simulink model "mars_rover_test_harness_chassis"  (R2025a)
settings: Solver=ode23t  StartTime=0.0  StopTime=30  FixedStep=1e-10  MaxStep=1e-1  RelTol=1e-3  AbsTol=1e-3  EnableMultiTasking=on
undefined symbols (not defined in the file): arm_q0, Control, L1, L2, L3, LS1, LS3, R1, R2, R3, Rover, RS1, RS3, X, Y, Z
libraries: sm_lib x119, nesl_utility x99, fl_lib x85, sdl_lib x20, ee_lib x10, mars_rover_lib x8, simulink x5, slpidlib x3, batteryecm_lib x2
(part 2 of 8)

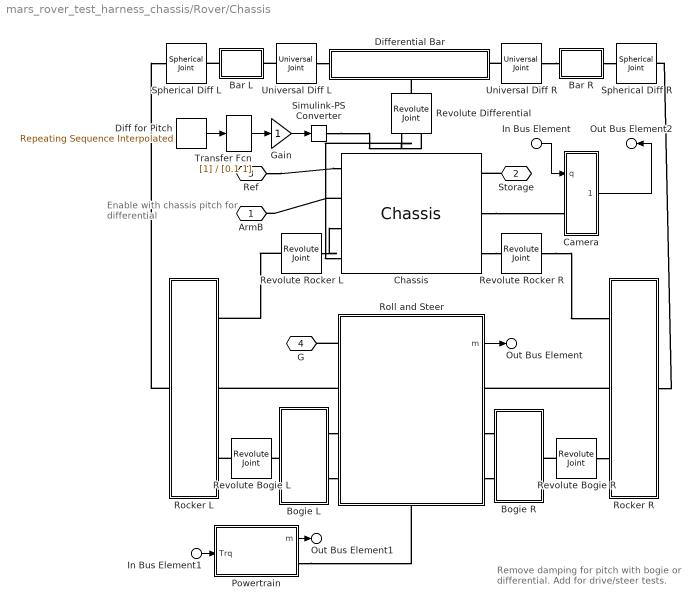
== system mars_rover_test_harness_chassis/Rover/Chassis ==
  note: Enable with chassis pitch for differential
  note: Remove damping for pitch with bogie or differential. Add for drive/steer tests.
  In Bus Element1 : Inport  PortName=Ctrl
  In Bus Element : Inport  PortName=Ctrl  Element=Camera
  Bar L : Subsystem
  Bar R : Subsystem
  Bogie L : Subsystem
      mask Display: image('mars_rover_terrain_chassis_bogiel.png');
  Bogie R : Subsystem
      mask Display: image('mars_rover_terrain_chassis_bogier.png');
  Camera : Subsystem
      mask Display: image('mars_rover_terrain_chassis_camera.png')
  Chassis : mars_rover_lib/Chassis  body_opc=1
  Diff for Pitch : simulink/Sources/Repeating Sequence Interpolated  OutValues=-0.5*[0 0 1 1 0 0 -1 -1 0 0]*5*pi/180.'  TimeValues=[0 2 4 7 9 11 13 16 18 20].'  LookUpMeth=Interpolation-Use End Values  tsamp=0.01  OutMin=[]  OutMax=[]  OutDataTypeStr=double  OutputDataTypeScalingMode=double  OutDataType=fixdt(0,8)  OutScaling=2^-10
  Differential Bar : Subsystem
      settings: PortSchema="{\"entries\":[{\"content\":{\"sides\":[{\"content\":{\"connectorIds\":[\"LConn1\"]},\"type\":\"ConnectorPlacement.EquallySpacedRectSide\",\"uuid\":\"221cdbde-9b85-4491-b488-ab21b8b80dc6\"},{\"content\":{\"connectorIds\":[\"RConn1\"],\"side\":\"RIGHT\"},\"type\":\"ConnectorPlacement.EquallySpacedRectSide\",\"uuid\":\"70e1e311-dd19-4389-b9b6-0ef8a1761d4a\"},{\"content\":{\"connectorIds\":[],\"side\":\"TOP\"},\"type\":\"ConnectorPlacement.EquallySpacedRectSide\",\"uuid\":\"5e164d53-108c-4bd4-88ac-8f7d3d652b3e\"},{\"content\":{\"connectorIds\":[\"RConn2\"],\"side\":\"BOTTOM\"},\"type\":\"ConnectorPlacement.EquallySpacedRectSide\",\"uuid\":\"f6e2e044-5d94-4f88-a007-0ec3cd9ea455\"}]},\"type\":\"ConnectorPlacement.EquallySpacedConnector\",\"uuid\":\"e7d2f355-3189-4eee-a2bf-989eae5d727a\"}],\"packageUris\":[\"http://schema.mathworks.com/mf0/Connector/R2020b\"],\"version\":\"1.0\"}"
      mask Display: image('mars_rover_terrain_chassis_diffarm.png');
  Gain : Gain
  Powertrain : Subsystem  Variant=on  VariantControlMode=label  VariantControl=Choice  LabelModeActiveChoice=Ideal  mask{popup_powertrain=Ideal}
      mask prompts: popup_powertrain "Powertrain Model"
      mask init:
      | set_param(gcb,'LabelModeActiveChoice',get_param(gcb,'popup_powertrain'));
      settings: AttributesFormatString=%<LabelModeActiveChoice>
      mask TypeOptions popup_powertrain: Ideal | Electrical
  Revolute Bogie L : sm_lib/Joints/Revolute Joint  JointMode=Normal  CompositeWrenchDir=FollowerOnBase  CompositeWrenchFrame=BaseFrame  SenseConstraintForce=off  SenseConstraintTorque=off  SenseTotalForce=off  SenseTotalTorque=off  PositionTargetSpecify=off  PositionTargetPriority=High  PositionTargetValue=0  PositionTargetValueUnits=deg  VelocityTargetSpecify=off  VelocityTargetPriority=High  VelocityTargetValue=0  VelocityTargetValueUnits=deg/s  EquilibriumPosition=0  EquilibriumPositionUnits=deg  SpringStiffness=0  SpringStiffnessUnits=N*m/deg  DampingCoefficient=1e3*0  DampingCoefficientUnits=N*m/(deg/s)  LowerLimitSpecify=off  LowerLimitBound=-90  LowerLimitBoundUnits=deg  LowerLimitStiffness=1e4  LowerLimitStiffnessUnits=N*m/deg  LowerLimitDamping=10  LowerLimitDampingUnits=N*m/(deg/s)  LowerLimitTransitionRegionWidth=0.1  LowerLimitTransitionRegionWidthUnits=deg  UpperLimitSpecify=off  UpperLimitBound=90  UpperLimitBoundUnits=deg  UpperLimitStiffness=1e4  UpperLimitStiffnessUnits=N*m/deg  UpperLimitDamping=10  UpperLimitDampingUnits=N*m/(deg/s)  UpperLimitTransitionRegionWidth=0.1  UpperLimitTransitionRegionWidthUnits=deg  TorqueActuationMode=NoTorque  MotionActuationMode=ComputedMotion  SensePosition=off  SenseVelocity=off  SenseAcceleration=off  SenseTorqueForce=off  SenseLowerLimitTorqueForce=off  SenseUpperLimitTorqueForce=off
  Revolute Bogie R : sm_lib/Joints/Revolute Joint  JointMode=Normal  CompositeWrenchDir=FollowerOnBase  CompositeWrenchFrame=BaseFrame  SenseConstraintForce=off  SenseConstraintTorque=off  SenseTotalForce=off  SenseTotalTorque=off  PositionTargetSpecify=off  PositionTargetPriority=High  PositionTargetValue=0  PositionTargetValueUnits=deg  VelocityTargetSpecify=off  VelocityTargetPriority=High  VelocityTargetValue=0  VelocityTargetValueUnits=deg/s  EquilibriumPosition=0  EquilibriumPositionUnits=deg  SpringStiffness=0  SpringStiffnessUnits=N*m/deg  DampingCoefficient=1e3*0  DampingCoefficientUnits=N*m/(deg/s)  LowerLimitSpecify=off  LowerLimitBound=-90  LowerLimitBoundUnits=deg  LowerLimitStiffness=1e4  LowerLimitStiffnessUnits=N*m/deg  LowerLimitDamping=10  LowerLimitDampingUnits=N*m/(deg/s)  LowerLimitTransitionRegionWidth=0.1  LowerLimitTransitionRegionWidthUnits=deg  UpperLimitSpecify=off  UpperLimitBound=90  UpperLimitBoundUnits=deg  UpperLimitStiffness=1e4  UpperLimitStiffnessUnits=N*m/deg  UpperLimitDamping=10  UpperLimitDampingUnits=N*m/(deg/s)  UpperLimitTransitionRegionWidth=0.1  UpperLimitTransitionRegionWidthUnits=deg  TorqueActuationMode=NoTorque  MotionActuationMode=ComputedMotion  SensePosition=off  SenseVelocity=off  SenseAcceleration=off  SenseTorqueForce=off  SenseLowerLimitTorqueForce=off  SenseUpperLimitTorqueForce=off
  Revolute Differential : sm_lib/Joints/Revolute Joint  JointMode=Normal  CompositeWrenchDir=FollowerOnBase  CompositeWrenchFrame=BaseFrame  SenseConstraintForce=off  SenseConstraintTorque=off  SenseTotalForce=off  SenseTotalTorque=off  PositionTargetSpecify=off  PositionTargetPriority=High  PositionTargetValue=45  PositionTargetValueUnits=deg  VelocityTargetSpecify=off  VelocityTargetPriority=High  VelocityTargetValue=1000  VelocityTargetValueUnits=deg/s  EquilibriumPosition=0  EquilibriumPositionUnits=deg  SpringStiffness=0  SpringStiffnessUnits=N*m/deg  DampingCoefficient=1e-3  DampingCoefficientUnits=N*m/(rad/s)  LowerLimitSpecify=off  LowerLimitBound=-90  LowerLimitBoundUnits=deg  LowerLimitStiffness=1e4  LowerLimitStiffnessUnits=N*m/deg  LowerLimitDamping=10  LowerLimitDampingUnits=N*m/(deg/s)  LowerLimitTransitionRegionWidth=0.1  LowerLimitTransitionRegionWidthUnits=deg  UpperLimitSpecify=off  UpperLimitBound=90  UpperLimitBoundUnits=deg  UpperLimitStiffness=1e4  UpperLimitStiffnessUnits=N*m/deg  UpperLimitDamping=10  UpperLimitDampingUnits=N*m/(deg/s)  UpperLimitTransitionRegionWidth=0.1  UpperLimitTransitionRegionWidthUnits=deg  TorqueActuationMode=ComputedTorque  MotionActuationMode=InputMotion  SensePosition=off  SenseVelocity=off  SenseAcceleration=off  SenseTorqueForce=off  SenseLowerLimitTorqueForce=off  SenseUpperLimitTorqueForce=off
  Revolute Rocker L : sm_lib/Joints/Revolute Joint  JointMode=Normal  CompositeWrenchDir=FollowerOnBase  CompositeWrenchFrame=BaseFrame  SenseConstraintForce=off  SenseConstraintTorque=off  SenseTotalForce=off  SenseTotalTorque=off  PositionTargetSpecify=on  PositionTargetPriority=Low  PositionTargetValue=90  PositionTargetValueUnits=deg  VelocityTargetSpecify=off  VelocityTargetPriority=High  VelocityTargetValue=5  VelocityTargetValueUnits=deg/s  EquilibriumPosition=0  EquilibriumPositionUnits=deg  SpringStiffness=0  SpringStiffnessUnits=N*m/deg  DampingCoefficient=1e3  DampingCoefficientUnits=N*m/(rad/s)  LowerLimitSpecify=off  LowerLimitBound=-90  LowerLimitBoundUnits=deg  LowerLimitStiffness=1e4  LowerLimitStiffnessUnits=N*m/deg  LowerLimitDamping=10  LowerLimitDampingUnits=N*m/(deg/s)  LowerLimitTransitionRegionWidth=0.1  LowerLimitTransitionRegionWidthUnits=deg  UpperLimitSpecify=off  UpperLimitBound=90  UpperLimitBoundUnits=deg  UpperLimitStiffness=1e4  UpperLimitStiffnessUnits=N*m/deg  UpperLimitDamping=10  UpperLimitDampingUnits=N*m/(deg/s)  UpperLimitTransitionRegionWidth=0.1  UpperLimitTransitionRegionWidthUnits=deg  TorqueActuationMode=NoTorque  MotionActuationMode=ComputedMotion  SensePosition=off  SenseVelocity=off  SenseAcceleration=off  SenseTorqueForce=off  SenseLowerLimitTorqueForce=off  SenseUpperLimitTorqueForce=off
  Revolute Rocker R : sm_lib/Joints/Revolute Joint  JointMode=Normal  CompositeWrenchDir=FollowerOnBase  CompositeWrenchFrame=BaseFrame  SenseConstraintForce=off  SenseConstraintTorque=off  SenseTotalForce=off  SenseTotalTorque=off  PositionTargetSpecify=on  PositionTargetPriority=Low  PositionTargetValue=-90  PositionTargetValueUnits=deg  VelocityTargetSpecify=off  VelocityTargetPriority=High  VelocityTargetValue=5  VelocityTargetValueUnits=deg/s  EquilibriumPosition=0  EquilibriumPositionUnits=deg  SpringStiffness=0  SpringStiffnessUnits=N*m/deg  DampingCoefficient=1e3  DampingCoefficientUnits=N*m/(rad/s)  LowerLimitSpecify=off  LowerLimitBound=-90  LowerLimitBoundUnits=deg  LowerLimitStiffness=1e4  LowerLimitStiffnessUnits=N*m/deg  LowerLimitDamping=10  LowerLimitDampingUnits=N*m/(deg/s)  LowerLimitTransitionRegionWidth=0.1  LowerLimitTransitionRegionWidthUnits=deg  UpperLimitSpecify=off  UpperLimitBound=90  UpperLimitBoundUnits=deg  UpperLimitStiffness=1e4  UpperLimitStiffnessUnits=N*m/deg  UpperLimitDamping=10  UpperLimitDampingUnits=N*m/(deg/s)  UpperLimitTransitionRegionWidth=0.1  UpperLimitTransitionRegionWidthUnits=deg  TorqueActuationMode=NoTorque  MotionActuationMode=ComputedMotion  SensePosition=off  SenseVelocity=off  SenseAcceleration=off  SenseTorqueForce=off  SenseLowerLimitTorqueForce=off  SenseUpperLimitTorqueForce=off
  Rocker L : Subsystem
      mask Display: image('mars_rover_terrain_chassis_rockerl.png');
  Rocker R : Subsystem
      mask Display: image('mars_rover_terrain_chassis_rockerr.png');
  Roll and Steer : Subsystem
      settings: PortSchema="{\"entries\":[{\"content\":{\"sides\":[{\"content\":{\"connectorIds\":[\"LConn1\",\"LConn2\",\"LConn3\",\"LConn4\"]},\"type\":\"ConnectorPlacement.EquallySpacedRectSide\",\"uuid\":\"a6cfb551-8d36-4b7b-a27d-860438164ad5\"},{\"content\":{\"connectorIds\":[\"Out1\",\"RConn1\",\"RConn2\",\"RConn3\"],\"side\":\"RIGHT\"},\"type\":\"ConnectorPlacement.EquallySpacedRectSide\",\"uuid\":\"63cd4134-c970-4875-8139-e10b865c9d5a\"},{\"content\":{\"connectorIds\":[],\"side\":\"TOP\"},\"type\":\"ConnectorPlacement.EquallySpacedRectSide\",\"uuid\":\"731de0f8-cd01-497c-8464-7874165ef328\"},{\"content\":{\"connectorIds\":[\"RConn4\"],\"side\":\"BOTTOM\"},\"type\":\"ConnectorPlacement.EquallySpacedRectSide\",\"uuid\":\"7e28c2ad-ee21-4cfa-8326-dce39ed3da54\"}]},\"type\":\"ConnectorPlacement.EquallySpacedConnector\",\"uuid\":\"7cc269d8-0205-4cd4-bd76-499a6cc04585\"}],\"packageUris\":[\"http://schema.mathworks.com/mf0/Connector/R2020b\"],\"version\":\"1.0\"}"
      mask Display: image('mars_rover_terrain_rollandsteer.png');
  Simulink-PS Converter : nesl_utility/Simulink-PS Converter  PhysicalDomain=network_engine_domain  SubClassName=ps_input  LeftPortType=input  RightPortType=output  PseudoPeriodic=off  Frequencies=[]  NoiseDistribution=none  NoiseParameters=[]  Unit=1  AffineConversion=off  FilteringAndDerivatives=filter  SimscapeFilterOrder=2  InputFilterTimeConstant=0.01  UdotUserProvided=0
  Spherical Diff L : sm_lib/Joints/Spherical Joint  JointMode=Normal  CompositeWrenchDir=FollowerOnBase  CompositeWrenchFrame=BaseFrame  SenseConstraintForce=off  SenseConstraintTorque=off  SenseTotalForce=off  SenseTotalTorque=off  PositionTargetSpecify=off  PositionTargetPriority=High  PositionTargetRotationMethod=None  PositionTargetFollAlignAxisA=+X  PositionTargetBaseAlignAxisA=+Y  PositionTargetFollAlignAxisB=+Y  PositionTargetBaseAlignAxisB=+Z  PositionTargetRotationStandardAxis=+Z  PositionTargetRotationAngle=0.0  PositionTargetRotationAngleUnits=deg  PositionTargetRotationArbitraryAxis=[0 0 1]  PositionTargetRotationSequenceAxes=FollowerAxes  PositionTargetRotationSequence=XYX  PositionTargetRotationSequenceAngles=[0 0 0]  PositionTargetRotationSequenceAnglesUnits=deg  PositionTargetRotationMatrix=[1 0 0; 0 1 0; 0 0 1]  PositionTargetQuaternion=[1 0 0 0]  VelocityTargetSpecify=off  VelocityTargetPriority=High  VelocityTargetValue=[0 0 0]  VelocityTargetValueUnits=deg/s  VelocityTargetInFollowerFrame=on  EqPosRotationMethod=None  EqPosFollAlignAxisA=+X  EqPosBaseAlignAxisA=+Y  EqPosFollAlignAxisB=+Y  EqPosBaseAlignAxisB=+Z  EqPosRotationStandardAxis=+Z  EqPosRotationAngle=0.0  EqPosRotationAngleUnits=deg  EqPosRotationArbitraryAxis=[0 0 1]  EqPosRotationSequenceAxes=FollowerAxes  EqPosRotationSequence=XYX  EqPosRotationSequenceAngles=[0 0 0]  EqPosRotationSequenceAnglesUnits=deg  EqPosRotationMatrix=[1 0 0; 0 1 0; 0 0 1]  EqPosQuaternion=[1 0 0 0]  SpringStiffness=0  SpringStiffnessUnits=N*m/deg  DampingCoefficient=1e-3  DampingCoefficientUnits=N*m/(deg/s)  LowerLimitSpecify=off  LowerLimitBound=15  LowerLimitBoundUnits=deg  LowerLimitStiffness=1e4  LowerLimitStiffnessUnits=N*m/deg  LowerLimitDamping=10  LowerLimitDampingUnits=N*m/(deg/s)  LowerLimitTransitionRegionWidth=0.1  LowerLimitTransitionRegionWidthUnits=deg  UpperLimitSpecify=off  UpperLimitBound=45  UpperLimitBoundUnits=deg  UpperLimitStiffness=1e4  UpperLimitStiffnessUnits=N*m/deg  UpperLimitDamping=10  UpperLimitDampingUnits=N*m/(deg/s)  UpperLimitTransitionRegionWidth=0.1  UpperLimitTransitionRegionWidthUnits=deg  TorqueActuationMode=NoTorque  ActuateTorqueX=off  ActuateTorqueY=off  ActuateTorqueZ=off  ActuateTorque=off  ActuationFrame=BaseFrame  SensePosition=off  SenseVelocityX=off  SenseVelocityY=off  SenseVelocityZ=off  SenseVelocity=off  SenseAccelerationX=off  SenseAccelerationY=off  SenseAccelerationZ=off  SenseAcceleration=off  SenseLowerLimitTorqueMag=off  SenseUpperLimitTorqueMag=off  SensingFrame=BaseFrame
  Spherical Diff R : sm_lib/Joints/Spherical Joint  JointMode=Normal  CompositeWrenchDir=FollowerOnBase  CompositeWrenchFrame=BaseFrame  SenseConstraintForce=off  SenseConstraintTorque=off  SenseTotalForce=off  SenseTotalTorque=off  PositionTargetSpecify=off  PositionTargetPriority=High  PositionTargetRotationMethod=None  PositionTargetFollAlignAxisA=+X  PositionTargetBaseAlignAxisA=+Y  PositionTargetFollAlignAxisB=+Y  PositionTargetBaseAlignAxisB=+Z  PositionTargetRotationStandardAxis=+Z  PositionTargetRotationAngle=0.0  PositionTargetRotationAngleUnits=deg  PositionTargetRotationArbitraryAxis=[0 0 1]  PositionTargetRotationSequenceAxes=FollowerAxes  PositionTargetRotationSequence=XYX  PositionTargetRotationSequenceAngles=[0 0 0]  PositionTargetRotationSequenceAnglesUnits=deg  PositionTargetRotationMatrix=[1 0 0; 0 1 0; 0 0 1]  PositionTargetQuaternion=[1 0 0 0]  VelocityTargetSpecify=off  VelocityTargetPriority=High  VelocityTargetValue=[0 0 0]  VelocityTargetValueUnits=deg/s  VelocityTargetInFollowerFrame=on  EqPosRotationMethod=None  EqPosFollAlignAxisA=+X  EqPosBaseAlignAxisA=+Y  EqPosFollAlignAxisB=+Y  EqPosBaseAlignAxisB=+Z  EqPosRotationStandardAxis=+Z  EqPosRotationAngle=0.0  EqPosRotationAngleUnits=deg  EqPosRotationArbitraryAxis=[0 0 1]  EqPosRotationSequenceAxes=FollowerAxes  EqPosRotationSequence=XYX  EqPosRotationSequenceAngles=[0 0 0]  EqPosRotationSequenceAnglesUnits=deg  EqPosRotationMatrix=[1 0 0; 0 1 0; 0 0 1]  EqPosQuaternion=[1 0 0 0]  SpringStiffness=0  SpringStiffnessUnits=N*m/deg  DampingCoefficient=1e-3  DampingCoefficientUnits=N*m/(deg/s)  LowerLimitSpecify=off  LowerLimitBound=15  LowerLimitBoundUnits=deg  LowerLimitStiffness=1e4  LowerLimitStiffnessUnits=N*m/deg  LowerLimitDamping=10  LowerLimitDampingUnits=N*m/(deg/s)  LowerLimitTransitionRegionWidth=0.1  LowerLimitTransitionRegionWidthUnits=deg  UpperLimitSpecify=off  UpperLimitBound=45  UpperLimitBoundUnits=deg  UpperLimitStiffness=1e4  UpperLimitStiffnessUnits=N*m/deg  UpperLimitDamping=10  UpperLimitDampingUnits=N*m/(deg/s)  UpperLimitTransitionRegionWidth=0.1  UpperLimitTransitionRegionWidthUnits=deg  TorqueActuationMode=NoTorque  ActuateTorqueX=off  ActuateTorqueY=off  ActuateTorqueZ=off  ActuateTorque=off  ActuationFrame=BaseFrame  SensePosition=off  SenseVelocityX=off  SenseVelocityY=off  SenseVelocityZ=off  SenseVelocity=off  SenseAccelerationX=off  SenseAccelerationY=off  SenseAccelerationZ=off  SenseAcceleration=off  SenseLowerLimitTorqueMag=off  SenseUpperLimitTorqueMag=off  SensingFrame=BaseFrame
  Transfer Fcn : TransferFcn  Denominator=[0.1 1]
  Universal Diff L : sm_lib/Joints/Universal Joint  JointMode=Normal  CompositeWrenchDir=FollowerOnBase  CompositeWrenchFrame=BaseFrame  SenseConstraintForce=off  SenseConstraintTorque=off  SenseTotalForce=off  SenseTotalTorque=off  RxPositionTargetSpecify=off  RxPositionTargetPriority=High  RxPositionTargetValue=0  RxPositionTargetValueUnits=deg  RxVelocityTargetSpecify=off  RxVelocityTargetPriority=High  RxVelocityTargetValue=0  RxVelocityTargetValueUnits=deg/s  RxEquilibriumPosition=0  RxEquilibriumPositionUnits=deg  RxSpringStiffness=0  RxSpringStiffnessUnits=N*m/deg  RxDampingCoefficient=0  RxDampingCoefficientUnits=N*m/(rad/s)  RxLowerLimitSpecify=off  RxLowerLimitBound=-90  RxLowerLimitBoundUnits=deg  RxLowerLimitStiffness=1e4  RxLowerLimitStiffnessUnits=N*m/deg  RxLowerLimitDamping=10  RxLowerLimitDampingUnits=N*m/(deg/s)  RxLowerLimitTransitionRegionWidth=0.1  RxLowerLimitTransitionRegionWidthUnits=deg  RxUpperLimitSpecify=off  RxUpperLimitBound=90  RxUpperLimitBoundUnits=deg  RxUpperLimitStiffness=1e4  RxUpperLimitStiffnessUnits=N*m/deg  RxUpperLimitDamping=10  RxUpperLimitDampingUnits=N*m/(deg/s)  RxUpperLimitTransitionRegionWidth=0.1  RxUpperLimitTransitionRegionWidthUnits=deg  RxTorqueActuationMode=NoTorque  RxMotionActuationMode=ComputedMotion  RxSensePosition=off  RxSenseVelocity=off  RxSenseAcceleration=off  RxSenseTorqueForce=off  RxSenseLowerLimitTorqueForce=off  RxSenseUpperLimitTorqueForce=off  RyPositionTargetSpecify=off  RyPositionTargetPriority=High  RyPositionTargetValue=0  RyPositionTargetValueUnits=deg  RyVelocityTargetSpecify=off  RyVelocityTargetPriority=High  RyVelocityTargetValue=0  RyVelocityTargetValueUnits=deg/s  RyEquilibriumPosition=0  RyEquilibriumPositionUnits=deg  RySpringStiffness=0  RySpringStiffnessUnits=N*m/deg  RyDampingCoefficient=0  RyDampingCoefficientUnits=N*m/(rad/s)  RyLowerLimitSpecify=off  RyLowerLimitBound=-90  RyLowerLimitBoundUnits=deg  RyLowerLimitStiffness=1e4  RyLowerLimitStiffnessUnits=N*m/deg  RyLowerLimitDamping=10  RyLowerLimitDampingUnits=N*m/(deg/s)  RyLowerLimitTransitionRegionWidth=0.1  RyLowerLimitTransitionRegionWidthUnits=deg  RyUpperLimitSpecify=off  RyUpperLimitBound=90  RyUpperLimitBoundUnits=deg  RyUpperLimitStiffness=1e4  RyUpperLimitStiffnessUnits=N*m/deg  RyUpperLimitDamping=10  RyUpperLimitDampingUnits=N*m/(deg/s)  RyUpperLimitTransitionRegionWidth=0.1  RyUpperLimitTransitionRegionWidthUnits=deg  RyTorqueActuationMode=NoTorque  RyMotionActuationMode=ComputedMotion  RySensePosition=off  RySenseVelocity=off  RySenseAcceleration=off  RySenseTorqueForce=off  RySenseLowerLimitTorqueForce=off  RySenseUpperLimitTorqueForce=off
  Universal Diff R : sm_lib/Joints/Universal Joint  JointMode=Normal  CompositeWrenchDir=FollowerOnBase  CompositeWrenchFrame=BaseFrame  SenseConstraintForce=off  SenseConstraintTorque=off  SenseTotalForce=off  SenseTotalTorque=off  RxPositionTargetSpecify=off  RxPositionTargetPriority=High  RxPositionTargetValue=0  RxPositionTargetValueUnits=deg  RxVelocityTargetSpecify=off  RxVelocityTargetPriority=High  RxVelocityTargetValue=0  RxVelocityTargetValueUnits=deg/s  RxEquilibriumPosition=0  RxEquilibriumPositionUnits=deg  RxSpringStiffness=0  RxSpringStiffnessUnits=N*m/deg  RxDampingCoefficient=0  RxDampingCoefficientUnits=N*m/(rad/s)  RxLowerLimitSpecify=off  RxLowerLimitBound=-90  RxLowerLimitBoundUnits=deg  RxLowerLimitStiffness=1e4  RxLowerLimitStiffnessUnits=N*m/deg  RxLowerLimitDamping=10  RxLowerLimitDampingUnits=N*m/(deg/s)  RxLowerLimitTransitionRegionWidth=0.1  RxLowerLimitTransitionRegionWidthUnits=deg  RxUpperLimitSpecify=off  RxUpperLimitBound=90  RxUpperLimitBoundUnits=deg  RxUpperLimitStiffness=1e4  RxUpperLimitStiffnessUnits=N*m/deg  RxUpperLimitDamping=10  RxUpperLimitDampingUnits=N*m/(deg/s)  RxUpperLimitTransitionRegionWidth=0.1  RxUpperLimitTransitionRegionWidthUnits=deg  RxTorqueActuationMode=NoTorque  RxMotionActuationMode=ComputedMotion  RxSensePosition=off  RxSenseVelocity=off  RxSenseAcceleration=off  RxSenseTorqueForce=off  RxSenseLowerLimitTorqueForce=off  RxSenseUpperLimitTorqueForce=off  RyPositionTargetSpecify=off  RyPositionTargetPriority=High  RyPositionTargetValue=0  RyPositionTargetValueUnits=deg  RyVelocityTargetSpecify=off  RyVelocityTargetPriority=High  RyVelocityTargetValue=0  RyVelocityTargetValueUnits=deg/s  RyEquilibriumPosition=0  RyEquilibriumPositionUnits=deg  RySpringStiffness=0  RySpringStiffnessUnits=N*m/deg  RyDampingCoefficient=0  RyDampingCoefficientUnits=N*m/(rad/s)  RyLowerLimitSpecify=off  RyLowerLimitBound=-90  RyLowerLimitBoundUnits=deg  RyLowerLimitStiffness=1e4  RyLowerLimitStiffnessUnits=N*m/deg  RyLowerLimitDamping=10  RyLowerLimitDampingUnits=N*m/(deg/s)  RyLowerLimitTransitionRegionWidth=0.1  RyLowerLimitTransitionRegionWidthUnits=deg  RyUpperLimitSpecify=off  RyUpperLimitBound=90  RyUpperLimitBoundUnits=deg  RyUpperLimitStiffness=1e4  RyUpperLimitStiffnessUnits=N*m/deg  RyUpperLimitDamping=10  RyUpperLimitDampingUnits=N*m/(deg/s)  RyUpperLimitTransitionRegionWidth=0.1  RyUpperLimitTransitionRegionWidthUnits=deg  RyTorqueActuationMode=NoTorque  RyMotionActuationMode=ComputedMotion  RySensePosition=off  RySenseVelocity=off  RySenseAcceleration=off  RySenseTorqueForce=off  RySenseLowerLimitTorqueForce=off  RySenseUpperLimitTorqueForce=off
  ArmB : PMIOPort  Side=Left
  Storage : PMIOPort  Port=2  Side=Left
  Ref : PMIOPort  Port=3  Side=Left
  G : PMIOPort  Port=4  Side=Left
  Out Bus Element : Outport  PortName=m  Element=Wheels
  Out Bus Element1 : Outport  PortName=m  Element=Powertrain
  Out Bus Element2 : Outport  PortName=m  Element=Camera
  wires:
  Roll and Steer/1(m) -> Out Bus Element/1
  In Bus Element1/1 -> Powertrain/1(Trq)
  Powertrain/1(m) -> Out Bus Element1/1
  In Bus Element/1 -> Camera/1(q)
  Camera/1(m) -> Out Bus Element2/1
  Diff for Pitch/1 -> Transfer Fcn/1
  Transfer Fcn/1 -> Gain/1
  Gain/1 -> Simulink-PS Converter/1
  connections:
  Ref/RConn1 -- Chassis/LConn1
  Revolute Rocker L/RConn1 -- Rocker L/RConn1
  Chassis/RConn3 -- Revolute Rocker R/LConn1
  Revolute Rocker L/LConn1 -- Chassis/LConn3
  Revolute Differential/LConn1 -- Chassis/LConn4
  Revolute Rocker R/RConn1 -- Rocker R/LConn1
  Revolute Differential/RConn1 -- Differential Bar/RConn2
  Rocker L/LConn1 -- Spherical Diff L/LConn1
  Rocker R/RConn1 -- Spherical Diff R/LConn1
  Rocker R/LConn2 -- Roll and Steer/RConn1
  Revolute Bogie R/LConn1 -- Rocker R/LConn3
  Chassis/LConn2 -- ArmB/RConn1
  Chassis/RConn2 -- Camera/LConn1
  Storage/RConn1 -- Chassis/RConn1
  Bogie L/RConn2 -- Roll and Steer/LConn4
  Bogie L/LConn1 -- Revolute Bogie L/RConn1
  Revolute Bogie R/RConn1 -- Bogie R/RConn1
  Roll and Steer/RConn2 -- Bogie R/LConn1
  Roll and Steer/RConn3 -- Bogie R/LConn2
  Roll and Steer/LConn1 -- G/RConn1
  Revolute Bogie L/LConn1 -- Rocker L/RConn3
  Roll and Steer/LConn2 -- Rocker L/RConn2
  Bogie L/RConn1 -- Roll and Steer/LConn3
  Powertrain/RConn1 -- Roll and Steer/RConn4
  Universal Diff L/RConn1 -- Bar L/LConn1
  Universal Diff L/LConn1 -- Differential Bar/LConn1
  Bar L/RConn1 -- Spherical Diff L/RConn1
  Universal Diff R/RConn1 -- Bar R/LConn1
  Universal Diff R/LConn1 -- Differential Bar/RConn1
  Bar R/RConn1 -- Spherical Diff R/RConn1
  Simulink-PS Converter/RConn1 -- Revolute Differential/LConn2

== system mars_rover_test_harness_chassis/Rover/Set Body Pitch ==
  note: Set switches to pitch body.
      |
      | Synchronize with differential movement if Pitch Differential is selected.
  Manual Switch : ManualSwitch
  Manual Switch1 : ManualSwitch  CurrentSetting=0
  No pitch : Constant  Value=0
  Pitch Bogie : simulink/Sources/Repeating Sequence Interpolated  OutValues=[0 0 1 1 0 0]*15*pi/180.'  TimeValues=[0 4 8 12 16 20].'  LookUpMeth=Interpolation-Use End Values  tsamp=0.01  OutMin=[]  OutMax=[]  OutDataTypeStr=double  OutputDataTypeScalingMode=double  OutDataType=fixdt(0,8)  OutScaling=2^-10
  Pitch Differential : simulink/Sources/Repeating Sequence Interpolated  OutValues=-0.5*[0 0 1 1 0 0 -1 -1 0 0]*12*pi/180.'  TimeValues=[0 2 4 7 9 11 13 16 18 20].'  LookUpMeth=Interpolation-Use End Values  tsamp=0.01  OutMin=[]  OutMax=[]  OutDataTypeStr=double  OutputDataTypeScalingMode=double  OutDataType=fixdt(0,8)  OutScaling=2^-10
  Revolute Joint : sm_lib/Joints/Revolute Joint  JointMode=Normal  CompositeWrenchDir=FollowerOnBase  CompositeWrenchFrame=BaseFrame  SenseConstraintForce=off  SenseConstraintTorque=off  SenseTotalForce=off  SenseTotalTorque=off  PositionTargetSpecify=off  PositionTargetPriority=High  PositionTargetValue=0  PositionTargetValueUnits=deg  VelocityTargetSpecify=off  VelocityTargetPriority=High  VelocityTargetValue=0  VelocityTargetValueUnits=deg/s  EquilibriumPosition=0  EquilibriumPositionUnits=deg  SpringStiffness=0  SpringStiffnessUnits=N*m/deg  DampingCoefficient=0  DampingCoefficientUnits=N*m/(deg/s)  LowerLimitSpecify=off  LowerLimitBound=-90  LowerLimitBoundUnits=deg  LowerLimitStiffness=1e4  LowerLimitStiffnessUnits=N*m/deg  LowerLimitDamping=10  LowerLimitDampingUnits=N*m/(deg/s)  LowerLimitTransitionRegionWidth=0.1  LowerLimitTransitionRegionWidthUnits=deg  UpperLimitSpecify=off  UpperLimitBound=90  UpperLimitBoundUnits=deg  UpperLimitStiffness=1e4  UpperLimitStiffnessUnits=N*m/deg  UpperLimitDamping=10  UpperLimitDampingUnits=N*m/(deg/s)  UpperLimitTransitionRegionWidth=0.1  UpperLimitTransitionRegionWidthUnits=deg  TorqueActuationMode=ComputedTorque  MotionActuationMode=InputMotion  SensePosition=off  SenseVelocity=off  SenseAcceleration=off  SenseTorqueForce=off  SenseLowerLimitTorqueForce=off  SenseUpperLimitTorqueForce=off
  Rigid Transform : sm_lib/Frames and Transforms/Rigid Transform  RotationMethod=StandardAxis  FollAlignAxisA=+X  BaseAlignAxisA=+Y  FollAlignAxisB=+Y  BaseAlignAxisB=+Z  RotationStandardAxis=+X  RotationAngle=-90  RotationAngleUnits=deg  RotationArbitraryAxis=[0 0 1]  RotationSequenceAxes=FollowerAxes  RotationSequence=XYX  RotationSequenceAngles=[0 0 0]  RotationSequenceAnglesUnits=deg  RotationMatrix=[1 0 0; 0 1 0; 0 0 1]  Quaternion=[1 0 0 0]  TranslationMethod=None  TranslationCartesianOffset=[0 0 0]  TranslationCartesianOffsetUnits=m  TranslationStandardAxis=+Z  TranslationStandardOffset=0  TranslationStandardOffsetUnits=m  TranslationROffset=0  TranslationROffsetUnits=m  TranslationThetaOffset=0  TranslationThetaOffsetUnits=deg  TranslationZOffset=0  TranslationZOffsetUnits=m
  Rigid Transform1 : sm_lib/Frames and Transforms/Rigid Transform  RotationMethod=StandardAxis  FollAlignAxisA=+X  BaseAlignAxisA=+Y  FollAlignAxisB=+Y  BaseAlignAxisB=+Z  RotationStandardAxis=+X  RotationAngle=-90  RotationAngleUnits=deg  RotationArbitraryAxis=[0 0 1]  RotationSequenceAxes=FollowerAxes  RotationSequence=XYX  RotationSequenceAngles=[0 0 0]  RotationSequenceAnglesUnits=deg  RotationMatrix=[1 0 0; 0 1 0; 0 0 1]  Quaternion=[1 0 0 0]  TranslationMethod=None  TranslationCartesianOffset=[0 0 0]  TranslationCartesianOffsetUnits=m  TranslationStandardAxis=+Z  TranslationStandardOffset=0  TranslationStandardOffsetUnits=m  TranslationROffset=0  TranslationROffsetUnits=m  TranslationThetaOffset=0  TranslationThetaOffsetUnits=deg  TranslationZOffset=0  TranslationZOffsetUnits=m
  Simulink-PS Converter : nesl_utility/Simulink-PS Converter  PhysicalDomain=network_engine_domain  SubClassName=ps_input  LeftPortType=input  RightPortType=output  PseudoPeriodic=off  Frequencies=[]  NoiseDistribution=none  NoiseParameters=[]  Unit=1  AffineConversion=off  FilteringAndDerivatives=filter  SimscapeFilterOrder=2  InputFilterTimeConstant=0.01  UdotUserProvided=0
  Transfer Fcn : TransferFcn  Denominator=[0.1 1]
  Transfer Fcn1 : TransferFcn  Denominator=[0.1 1]
  B : PMIOPort  Side=Left
  F : PMIOPort  Port=2  Side=Right
  wires:
  Pitch Bogie/1 -> Transfer Fcn/1
  Transfer Fcn1/1 -> Manual Switch/2
  Pitch Differential/1 -> Transfer Fcn1/1
  Transfer Fcn/1 -> Manual Switch/1
  Manual Switch/1 -> Manual Switch1/1
  Manual Switch1/1 -> Simulink-PS Converter/1
  No pitch/1 -> Manual Switch1/2
  connections:
  Rigid Transform/RConn1 -- Revolute Joint/LConn1
  Rigid Transform1/RConn1 -- Revolute Joint/RConn1
  Rigid Transform1/LConn1 -- F/RConn1
  Rigid Transform/LConn1 -- B/RConn1
  Simulink-PS Converter/RConn1 -- Revolute Joint/LConn2

== system mars_rover_test_harness_chassis/Control/Arm Control/Bus to Vec q ==
  B : Inport
  Bus Selector : BusSelector  OutputSignals=q.q1,q.q2,q.q3,q.q4,q.q5,q.q6
  Mux : Mux  Inputs=6
  V : Outport
  wires:
  Bus Selector/6 -> Mux/6  "<q6>"
  Bus Selector/4 -> Mux/4  "<q4>"
  Mux/1 -> V/1
  B/1 -> Bus Selector/1
  Bus Selector/1 -> Mux/1  "<q1>"
  Bus Selector/3 -> Mux/3  "<q3>"
  Bus Selector/2 -> Mux/2  "<q2>"
  Bus Selector/5 -> Mux/5  "<q5>"

== system mars_rover_test_harness_chassis/Control/Arm Control/Vec to Bus q ==
  V : Inport
  Bus Creator : BusCreator  Inputs=6
  Demux : Demux  Outputs=6
  B : Outport
  wires:
  Demux/3 -> Bus Creator/3  "q3"
  Bus Creator/1 -> B/1
  V/1 -> Demux/1
  Demux/4 -> Bus Creator/4  "q4"
  Demux/1 -> Bus Creator/1  "q1"
  Demux/6 -> Bus Creator/6  "q6"
  Demux/2 -> Bus Creator/2  "q2"
  Demux/5 -> Bus Creator/5  "q5"

== system mars_rover_test_harness_chassis/Control/Arm Control/Vec to Bus trq ==
  V : Inport
  Bus Creator : BusCreator  Inputs=6
  Demux : Demux  Outputs=6
  B : Outport
  wires:
  Demux/5 -> Bus Creator/5  "t5"
  Demux/2 -> Bus Creator/2  "t2"
  Demux/6 -> Bus Creator/6  "t6"
  Demux/1 -> Bus Creator/1  "t1"
  Demux/4 -> Bus Creator/4  "t4"
  V/1 -> Demux/1
  Bus Creator/1 -> B/1
  Demux/3 -> Bus Creator/3  "t3"

== system mars_rover_test_harness_chassis/Control/Chassis Control/Ackerman Steer Angle ==
  note: ROC: Radius of Curvature
      | A3: Axle 3
      | L3: Rear Left Wheel
      | R3: Rear Right Wheel
  AtGoal : Inport
  Delta : Inport  Port=2
  Ackerman Steering Angle Formulation : MATLAB Function  TreatAsAtomicUnit=on
  Clock1 : Clock
  Constant : Constant  Value=Rover.Chassis.Length/2
  Constant3 : Constant  Value=0
  Constant4 : Constant  Value=Rover.Chassis.Width
  Gain3 : Gain  Gain=-1
  Gain4 : Gain  Gain=-1
  Hold Steer at Goal : Subsystem  TreatAsAtomicUnit=on
  Mux : Mux
  NOT : Logic  Operator=NOT  IconShape=distinctive  AllPortsSameDT=off  OutDataTypeStr=boolean
  Saturation{1..4} (4 alike) : Saturate  UpperLimit=60  LowerLimit=-60
  Scope : Scope  NumInputPorts=3
      settings: ActiveDisplayYMinimum=-35.60933  ActiveDisplayYMaximum=51.25577  DataLoggingVariableName=ScopeData2
  Switch2 : Switch  Criteria=u2 > Threshold  Threshold=1  SaturateOnIntegerOverflow=off  InputSameDT=off
  AckSteerAngs : Outport
  A3 ROC : Outport  Port=2
  L3ROC : Outport  Port=3
  R3ROC : Outport  Port=4
  wires:
  Delta/1 -> Switch2/1
  Ackerman Steering Angle Formulation/2(qSteerR3) -> Scope/3, Saturation3/1, Gain4/1
  Ackerman Steering Angle Formulation/5(R_R) -> R3ROC/1
  Saturation4/1 -> Mux/4  "R1"
  Saturation1/1 -> Mux/2  "L1"
  Hold Steer at Goal/1(d_h) -> Scope/1, Ackerman Steering Angle Formulation/1(delta)
  Ackerman Steering Angle Formulation/1(qSteerL3) -> Scope/2, Saturation2/1, Gain3/1
  Constant/1 -> Ackerman Steering Angle Formulation/2(L)
  Saturation3/1 -> Mux/3  "R3"
  Mux/1 -> AckSteerAngs/1
  Clock1/1 -> Switch2/2
  Switch2/1 -> Hold Steer at Goal/1(d)
  Gain4/1 -> Saturation4/1
  Saturation2/1 -> Mux/1  "L3"
  Constant4/1 -> Ackerman Steering Angle Formulation/3(d)
  Gain3/1 -> Saturation1/1
  Ackerman Steering Angle Formulation/4(L_R) -> L3ROC/1
  Ackerman Steering Angle Formulation/3(R) -> A3 ROC/1
  Constant3/1 -> Switch2/3
  AtGoal/1 -> NOT/1
  NOT/1 -> Hold Steer at Goal/Enable

== system mars_rover_test_harness_chassis/Control/Chassis Control/Steering Controller ==
  Meas : Inport
  qSteerWhl : Inport  Port=2
  RoverAtGoal : Inport  Port=3
  Add : Sum  Inputs=+-
  Bus to Vec : Subsystem
  Check Difference : Subsystem
  Constant : Constant  Value=[Kp Ki]
  Constant1 : Constant  Value=[10 1 ]
  Constant2 : Constant  Value=Kd
  Constant3 : Constant  Value=N
  Demux : Demux  Outputs=2
  Demux1 : Demux
  Filter qMeas : Subsystem  mask(First-order lag supporting vector signals){b=[1 1 1 1]*Ts_Measq, x_initial=[0 0 0 0]}
      mask prompts: b "Filter time constant"; x_initial "Initial output"
      mask help: Models a lag of the form 1/(b*s+1) where s is the Laplace operator.
  Filter qTarget : Subsystem  mask(First-order lag supporting vector signals){b=[1 1 1 1]*Ts_Targetq, x_initial=[0 0 0 0]}
      mask prompts: b "Filter time constant"; x_initial "Initial output"
      mask help: Models a lag of the form 1/(b*s+1) where s is the Laplace operator.
  PID Controller : slpidlib/PID Controller  Controller=PID  Form=Parallel  TimeDomain=Continuous-time  UseExternalTs=off  SampleTime=-1  IntegratorMethod=Forward Euler  FilterMethod=Forward Euler  ControllerParametersSource=external  P=1  I=0  UseKiTs=off  D=0  UseExternalDerivativeSource=off  N=10  UseFilter=on  TunerSelectOption=Transfer Function Based (PID Tuner App)  InitialConditionSource=internal  InitialConditionForIntegrator=0  InitialConditionForFilter=0  DifferentiatorICPrevScaledInput=0  ExternalReset=none  TrackingMode=off  Kt=1  LimitOutput=on  SatLimitsSource=internal  UpperSaturationLimit=trq_max_pos  LowerSaturationLimit=trq_max_neg  LinearizeAsGain=on  AntiWindupMode=none  Kb=1  LimitIntegrator=off  UpperIntegratorSaturationLimit=inf  LowerIntegratorSaturationLimit=-inf  POutMin=[]  POutMax=[]  IOutMin=[]  IOutMax=[]  DOutMin=[]  DOutMax=[]  NOutMin=[]  NOutMax=[]  SumOutMin=[]  SumOutMax=[]  SaturationOutMin=[]  SaturationOutMax=[]  PParamMin=[]  PParamMax=[]  IParamMin=[]  IParamMax=[]  DParamMin=[]  DParamMax=[]  NParamMin=[]  NParamMax=[]  KbParamMin=[]  KbParamMax=[]  KtParamMin=[]  KtParamMax=[]  KbOutMin=[]  KbOutMax=[]  KtOutMin=[]  KtOutMax=[]  IntegratorOutMin=[]  IntegratorOutMax=[]  FilterOutMin=[]  FilterOutMax=[]  SumI1OutMin=[]  SumI1OutMax=[]  SumI2OutMin=[]  SumI2OutMax=[]  SumI3OutMin=[]  SumI3OutMax=[]  SumI4OutMin=[]  SumI4OutMax=[]  SumDOutMin=[]  SumDOutMax=[]  DifferentiatorOutMin=[]  DifferentiatorOutMax=[]  FilterDiffOutCoefMin=[]  FilterDiffOutCoefMax=[]  ReciprocalOutMin=[]  ReciprocalOutMax=[]  SumDenOutMin=[]  SumDenOutMax=[]  SumNumOutMin=[]  SumNumOutMax=[]  DivideOutMin=[]  DivideOutMax=[]  UdiffTsProdOutMin=[]  UdiffTsProdOutMax=[]  NTsProdOutMin=[]  NTsProdOutMax=[]  UintegralTsProdOutMin=[]  UintegralTsProdOutMax=[]  UngainTsProdOutMin=[]  UngainTsProdOutMax=[]  ClampingZeroOutDataTypeStr=Inherit: Inherit via back propagation  ClampingZeroOutMin=[]  ClampingZeroOutMax=[]  FilterDenConstantOutDataTypeStr=Inherit: Inherit via back propagation  FilterDenConstantOutMin=[]  FilterDenConstantOutMax=[]  PCopyOutDataTypeStr=Inherit: Inherit via back propagation  PCopyOutMin=[]  PCopyOutMax=[]  NCopyOutDataTypeStr=Inherit: Inherit via back propagation  NCopyOutMin=[]  NCopyOutMax=[]  IntegratorContinuousStateAttributes=''  IntegratorStateMustResolveToSignalObject=off  IntegratorRTWStateStorageClass=Auto  FilterContinuousStateAttributes=''  FilterStateMustResolveToSignalObject=off  FilterRTWStateStorageClass=Auto  ParallelPVariant=ExternalParameters  IdealPVariant=Disabled  IVariant=ExternalParameters  DVariant=ExternalParameters  IntegratorVariant=Continuous  SatVariant=Enabled  AWVariant=Passthrough  PCopyVariant=Disabled  TRVariant=Disabled  FdbkBlocksVariant=Forward  IdealPFdbkVariant=Disabled  SatFdbkVariant=Disabled  DerivativeFilterVariant=ContFilter  NVariant=ExternalParameters  NCopyVariant=Disabled  FilterICVariant=InternalICsFilter  IntegratorICVariant=InternalICs  ExternalResetVariant=Disabled  TRSumVariant=Passthrough  SumFdbkVariant=Disabled  SumVariant=Sum_PID  TsampFilterVariant=InternalTs  TsampNgainVariant=Passthrough  TsampIntegralVariant=Disabled_SignalSpec  ExternalSaturationOutDataTypeStr=Inherit: Same as second input  DerivativeSourceVariant=ErrorSignal  PreIntVariant=InternalPreInt
  Scope : Scope  NumInputPorts=4
      settings: ActiveDisplayYMinimum=-152.13979  ActiveDisplayYMaximum=38.47588
  Scope1 : Scope  NumInputPorts=4
      settings: ActiveDisplayYMinimum=-2.45349  ActiveDisplayYMaximum=1.54302  DataLoggingVariableName=ScopeData5
  Switch : Switch  Criteria=u2 > Threshold  SaturateOnIntegerOverflow=off  InputSameDT=off
  trq : Outport
  wires:
  PID Controller/1 -> trq/1
  qSteerWhl/1 -> Filter qTarget/1(In)
  Add/1 -> PID Controller/1, Demux1/1
  RoverAtGoal/1 -> Switch/2
  Constant1/1 -> Switch/1
  Demux/1 -> PID Controller/2
  Demux/2 -> PID Controller/3
  Constant/1 -> Switch/3
  Switch/1 -> Demux/1
  Meas/1 -> Bus to Vec/1(B)
  Bus to Vec/1(V) -> Filter qMeas/1(In)
  Check Difference/1(Out1) -> Scope/1
  Check Difference/2(Out2) -> Scope/2
  Check Difference/3(Out3) -> Scope/3
  Check Difference/4(Out4) -> Scope/4
  Constant2/1 -> PID Controller/4
  Filter qMeas/1(Out) -> Check Difference/2(In2), Add/2
  Filter qTarget/1(Out) -> Add/1, Check Difference/1(In1)
  Demux1/1 -> Scope1/1
  Demux1/2 -> Scope1/2
  Demux1/3 -> Scope1/3
  Demux1/4 -> Scope1/4
  Constant3/1 -> PID Controller/5

== system mars_rover_test_harness_chassis/Control/Chassis Control/Vec to Bus SteerTrq ==
  V : Inport
  Bus Creator : BusCreator  Inputs=4
  Demux : Demux
  B : Outport
  wires:
  Demux/3 -> Bus Creator/3  "R3"
  Bus Creator/1 -> B/1
  V/1 -> Demux/1
  Demux/4 -> Bus Creator/4  "R1"
  Demux/1 -> Bus Creator/1  "L3"
  Demux/2 -> Bus Creator/2  "L1"

== system mars_rover_test_harness_chassis/Control/Chassis Control/Vec to Bus qSteer ==
  V : Inport
  Bus Creator : BusCreator  Inputs=4
  Demux : Demux
  B : Outport
  wires:
  Demux/2 -> Bus Creator/2  "L1"
  Demux/4 -> Bus Creator/4  "R1"
  Demux/3 -> Bus Creator/3  "R3"
  Demux/1 -> Bus Creator/1  "L3"
  Bus Creator/1 -> B/1
  V/1 -> Demux/1

== system mars_rover_test_harness_chassis/Control/Chassis Control/Vec to Bus trq ==
  V : Inport
  Bus Creator : BusCreator  Inputs=6
  Demux : Demux  Outputs=6
  B : Outport
  wires:
  Demux/5 -> Bus Creator/5  "R2"
  Demux/2 -> Bus Creator/2  "L2"
  Demux/6 -> Bus Creator/6  "R3"
  Demux/1 -> Bus Creator/1  "L1"
  Demux/4 -> Bus Creator/4  "R1"
  V/1 -> Demux/1
  Bus Creator/1 -> B/1
  Demux/3 -> Bus Creator/3  "L3"

== system mars_rover_test_harness_chassis/Control/Chassis Control/Vec to Bus wWhl ==
  V : Inport
  Bus Creator : BusCreator  Inputs=6
  Demux : Demux  Outputs=6
  B : Outport
  wires:
  V/1 -> Demux/1
  Bus Creator/1 -> B/1
  Demux/1 -> Bus Creator/1  "L1"
  Demux/3 -> Bus Creator/3  "L3"
  Demux/4 -> Bus Creator/4  "R1"
  Demux/2 -> Bus Creator/2  "L2"
  Demux/5 -> Bus Creator/5  "R2"
  Demux/6 -> Bus Creator/6  "R3"

== system mars_rover_test_harness_chassis/Control/Chassis Control/Wheel Speed Controller ==
  Meas : Inport
  StopAtGoal : Inport  Port=2
  wTarget : Inport  Port=3
  Add3 : Sum  Inputs=+-
  Bus to Vec : Subsystem
  Constant : Constant  Value=[Kp,Ki]
  Constant1 : Constant  Value=[5000 100]
  Constant2 : Constant  Value=Kd
  Constant3 : Constant  Value=N
  Demux : Demux  Outputs=2
  Filter wMeas : Subsystem  mask(First-order lag supporting vector signals){b=[1 1 1 1 1 1]*Ts_Measw, x_initial=[0 0 0 0 0 0]}
      mask prompts: b "Filter time constant"; x_initial "Initial output"
      mask help: Models a lag of the form 1/(b*s+1) where s is the Laplace operator.
  Filter wTarget : Subsystem  mask(First-order lag supporting vector signals){b=[1 1 1 1 1 1]*Ts_Targetw, x_initial=[0 0 0 0 0 0]}
      mask prompts: b "Filter time constant"; x_initial "Initial output"
      mask help: Models a lag of the form 1/(b*s+1) where s is the Laplace operator.
  PID Controller : slpidlib/PID Controller  Controller=PID  Form=Parallel  TimeDomain=Continuous-time  UseExternalTs=off  SampleTime=-1  IntegratorMethod=Forward Euler  FilterMethod=Forward Euler  ControllerParametersSource=external  P=1  I=0  UseKiTs=off  D=0  UseExternalDerivativeSource=off  N=100  UseFilter=on  TunerSelectOption=Transfer Function Based (PID Tuner App)  InitialConditionSource=internal  InitialConditionForIntegrator=0  InitialConditionForFilter=0  DifferentiatorICPrevScaledInput=0  ExternalReset=none  TrackingMode=off  Kt=1  LimitOutput=off  SatLimitsSource=internal  UpperSaturationLimit=inf  LowerSaturationLimit=-inf  LinearizeAsGain=on  AntiWindupMode=none  Kb=1  LimitIntegrator=off  UpperIntegratorSaturationLimit=inf  LowerIntegratorSaturationLimit=-inf  POutMin=[]  POutMax=[]  IOutMin=[]  IOutMax=[]  DOutMin=[]  DOutMax=[]  NOutMin=[]  NOutMax=[]  SumOutMin=[]  SumOutMax=[]  SaturationOutMin=[]  SaturationOutMax=[]  PParamMin=[]  PParamMax=[]  IParamMin=[]  IParamMax=[]  DParamMin=[]  DParamMax=[]  NParamMin=[]  NParamMax=[]  KbParamMin=[]  KbParamMax=[]  KtParamMin=[]  KtParamMax=[]  KbOutMin=[]  KbOutMax=[]  KtOutMin=[]  KtOutMax=[]  IntegratorOutMin=[]  IntegratorOutMax=[]  FilterOutMin=[]  FilterOutMax=[]  SumI1OutMin=[]  SumI1OutMax=[]  SumI2OutMin=[]  SumI2OutMax=[]  SumI3OutMin=[]  SumI3OutMax=[]  SumI4OutMin=[]  SumI4OutMax=[]  SumDOutMin=[]  SumDOutMax=[]  DifferentiatorOutMin=[]  DifferentiatorOutMax=[]  FilterDiffOutCoefMin=[]  FilterDiffOutCoefMax=[]  ReciprocalOutMin=[]  ReciprocalOutMax=[]  SumDenOutMin=[]  SumDenOutMax=[]  SumNumOutMin=[]  SumNumOutMax=[]  DivideOutMin=[]  DivideOutMax=[]  UdiffTsProdOutMin=[]  UdiffTsProdOutMax=[]  NTsProdOutMin=[]  NTsProdOutMax=[]  UintegralTsProdOutMin=[]  UintegralTsProdOutMax=[]  UngainTsProdOutMin=[]  UngainTsProdOutMax=[]  ClampingZeroOutDataTypeStr=Inherit: Inherit via back propagation  ClampingZeroOutMin=[]  ClampingZeroOutMax=[]  FilterDenConstantOutDataTypeStr=Inherit: Inherit via back propagation  FilterDenConstantOutMin=[]  FilterDenConstantOutMax=[]  PCopyOutDataTypeStr=Inherit: Inherit via back propagation  PCopyOutMin=[]  PCopyOutMax=[]  NCopyOutDataTypeStr=Inherit: Inherit via back propagation  NCopyOutMin=[]  NCopyOutMax=[]  IntegratorContinuousStateAttributes=''  IntegratorStateMustResolveToSignalObject=off  IntegratorRTWStateStorageClass=Auto  FilterContinuousStateAttributes=''  FilterStateMustResolveToSignalObject=off  FilterRTWStateStorageClass=Auto  ParallelPVariant=ExternalParameters  IdealPVariant=Disabled  IVariant=ExternalParameters  DVariant=ExternalParameters  IntegratorVariant=Continuous  SatVariant=Disabled  AWVariant=Passthrough  PCopyVariant=Disabled  TRVariant=Disabled  FdbkBlocksVariant=Forward  IdealPFdbkVariant=Disabled  SatFdbkVariant=Disabled  DerivativeFilterVariant=ContFilter  NVariant=ExternalParameters  NCopyVariant=Disabled  FilterICVariant=InternalICsFilter  IntegratorICVariant=InternalICs  ExternalResetVariant=Disabled  TRSumVariant=Passthrough  SumFdbkVariant=Disabled  SumVariant=Sum_PID  TsampFilterVariant=InternalTs  TsampNgainVariant=Passthrough  TsampIntegralVariant=Disabled_SignalSpec  ExternalSaturationOutDataTypeStr=Inherit: Same as second input  DerivativeSourceVariant=ErrorSignal  PreIntVariant=InternalPreInt
  Saturation : Saturate  UpperLimit=trq_max_pos  LowerLimit=trq_max_neg
  Switch : Switch  Criteria=u2 > Threshold  SaturateOnIntegerOverflow=off  InputSameDT=off
  trq : Outport
  wires:
  Switch/1 -> Demux/1
  Constant/1 -> Switch/3
  Constant1/1 -> Switch/1
  Demux/2 -> PID Controller/3
  Demux/1 -> PID Controller/2
  StopAtGoal/1 -> Switch/2
  PID Controller/1 -> Saturation/1
  Meas/1 -> Bus to Vec/1(B)
  Add3/1 -> PID Controller/1
  Saturation/1 -> trq/1
  Bus to Vec/1(V) -> Filter wMeas/1(In)
  wTarget/1 -> Filter wTarget/1(In)
  Constant2/1 -> PID Controller/4
  Constant3/1 -> PID Controller/5
  Filter wMeas/1(Out) -> Add3/2
  Filter wTarget/1(Out) -> Add3/1

== system mars_rover_test_harness_chassis/Rover/Chassis/Bar L ==
  Connecting Bar L : sm_lib/Body Elements/Brick Solid  BrickDimensions=[1 20.000000607487117 1]  BrickDimensionsUnits=cm  ExportEntireGeometry=off  InertiaType=CalculateFromGeometry  BasedOnType=Density  Density=2700  DensityUnits=kg/m^3  Mass=3  MassUnits=kg  CenterOfMass=[0 0 0]  CenterOfMassUnits=m  MomentsOfInertia=[1 1 1]  MomentsOfInertiaUnits=kg*m^2  ProductsOfInertia=[0 0 0]  ProductsOfInertiaUnits=kg*m^2  GraphicType=FromGeometry  MarkerShape=Sphere  MarkerSize=10  GraphicVisPropType=SimpleVisualProperties  GraphicDiffuseColor=[0.5 0.5 0.5]  GraphicOpacity=1.0  GraphicSpecularColor=[0.5 0.5 0.5 1.0]  GraphicAmbientColor=[0.15 0.15 0.15 1.0]  GraphicEmissiveColor=[0.0 0.0 0.0 1.0]  GraphicShininess=75  DoExposeReferenceFrame=off  SerializedFrames=<Frames><Frame><Id>Frame1</Id><Value><Name>F1</Name><Origin><Source>GeometricFeature</Source><FeatureName>-y surface</FeatureName></Origin><PrimaryAxis><DefinedDirection>+Z</DefinedDirection><Source>ReferenceFrame</Source><SourceDirection>+Z</SourceDirection><FeatureName></FeatureName></PrimaryAxis><SecondaryAxis><DefinedDirection>+X</DefinedDirection><Source>ReferenceFrame</Source><SourceDirection>+X</SourceDirection><FeatureName></FeatureName></SecondaryAxis></Value></Frame><Frame><Id>Frame2</Id><Value><Name>F2</Name><Origin><Source>GeometricFeature</Source><FeatureName>+y surface</FeatureName></Origin><PrimaryAxis><DefinedDirection>+Z</DefinedDirection><Source>ReferenceFrame</Source><SourceDirection>+X</SourceDirection><FeatureName></FeatureName></PrimaryAxis><SecondaryAxis><DefinedDirection>+X</DefinedDirection><Source>ReferenceFrame</Source><SourceDirection>-Y</SourceDirection><FeatureName></FeatureName></SecondaryAxis></Value></Frame></Frames>
  Rigid Transform2 : sm_lib/Frames and Transforms/Rigid Transform  RotationMethod=StandardAxis  FollAlignAxisA=+X  BaseAlignAxisA=+Y  FollAlignAxisB=+Y  BaseAlignAxisB=+Z  RotationStandardAxis=+X  RotationAngle=90  RotationAngleUnits=deg  RotationArbitraryAxis=[0 0 1]  RotationSequenceAxes=FollowerAxes  RotationSequence=XYX  RotationSequenceAngles=[0 0 0]  RotationSequenceAnglesUnits=deg  RotationMatrix=[1 0 0; 0 1 0; 0 0 1]  Quaternion=[1 0 0 0]  TranslationMethod=None  TranslationCartesianOffset=[0 0 0]  TranslationCartesianOffsetUnits=m  TranslationStandardAxis=+Z  TranslationStandardOffset=0  TranslationStandardOffsetUnits=m  TranslationROffset=0  TranslationROffsetUnits=m  TranslationThetaOffset=0  TranslationThetaOffsetUnits=deg  TranslationZOffset=0  TranslationZOffsetUnits=m
  Rigid Transform4 : sm_lib/Frames and Transforms/Rigid Transform  RotationMethod=None  FollAlignAxisA=+X  BaseAlignAxisA=+Y  FollAlignAxisB=+Y  BaseAlignAxisB=+Z  RotationStandardAxis=+X  RotationAngle=180  RotationAngleUnits=deg  RotationArbitraryAxis=[0 0 1]  RotationSequenceAxes=FollowerAxes  RotationSequence=XYX  RotationSequenceAngles=[0 0 0]  RotationSequenceAnglesUnits=deg  RotationMatrix=[1 0 0; 0 1 0; 0 0 1]  Quaternion=[1 0 0 0]  TranslationMethod=None  TranslationCartesianOffset=[0 0 0]  TranslationCartesianOffsetUnits=m  TranslationStandardAxis=+Z  TranslationStandardOffset=0  TranslationStandardOffsetUnits=m  TranslationROffset=0  TranslationROffsetUnits=m  TranslationThetaOffset=0  TranslationThetaOffsetUnits=deg  TranslationZOffset=0  TranslationZOffsetUnits=m
  B : PMIOPort  Side=Left
  F : PMIOPort  Port=2  Side=Right
  connections:
  Rigid Transform4/LConn1 -- Rigid Transform2/LConn1
  Connecting Bar L/LConn1 -- Rigid Transform4/RConn1
  Rigid Transform2/RConn1 -- B/RConn1
  Connecting Bar L/RConn1 -- F/RConn1
